simulink model "hw3_model"  (R2024b)
settings: Solver=ode4  StartTime=0.0  StopTime=120.0  FixedStep=0.05  RelTol=1e-3
undefined symbols (not defined in the file): k, L, v, waypoints
settings Model: Creator=Atakan  LastModifiedBy=Atakan

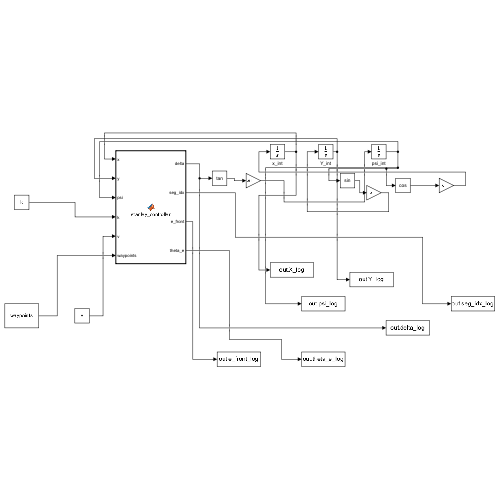
[thumbnail: Simulink's stored preview of the top-level diagram]
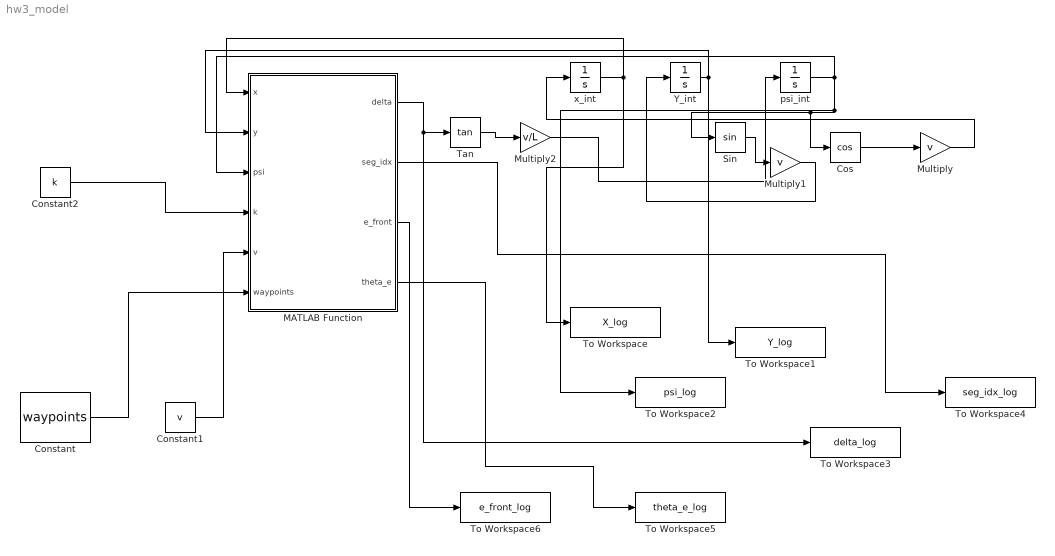
== system hw3_model ==
  Constant : Constant  Value=waypoints
  Constant1 : Constant  Value=v
  Constant2 : Constant  Value=k
  Cos : Trigonometry  Operator=cos
  MATLAB Function : MATLAB Function  TreatAsAtomicUnit=on  SystemSampleTime=0.05
  Multiply : Gain  Gain=v
  Multiply1 : Gain  Gain=v
  Multiply2 : Gain  Gain=v/L
  Sin : Trigonometry
  Tan : Trigonometry  Operator=tan
  To Workspace : ToWorkspace  VariableName=X_log  SaveFormat=Timeseries  SampleTime=-1
  To Workspace1 : ToWorkspace  VariableName=Y_log  SaveFormat=Timeseries  SampleTime=-1
  To Workspace2 : ToWorkspace  VariableName=psi_log  SaveFormat=Timeseries  SampleTime=-1
  To Workspace3 : ToWorkspace  VariableName=delta_log  SaveFormat=Timeseries  SampleTime=-1
  To Workspace4 : ToWorkspace  VariableName=seg_idx_log  SaveFormat=Timeseries  SampleTime=-1
  To Workspace5 : ToWorkspace  VariableName=theta_e_log  SaveFormat=Timeseries  SampleTime=-1
  To Workspace6 : ToWorkspace  VariableName=e_front_log  SaveFormat=Timeseries  SampleTime=-1
  Y_int : Integrator
  psi_int : Integrator  InitialCondition=atan2(5,10)
  x_int : Integrator
  wires:
  psi_int/1 -> To Workspace2/1, Sin/1, Cos/1, MATLAB Function/3(psi)
  Cos/1 -> Multiply/1
  Multiply/1 -> x_int/1
  Sin/1 -> Multiply1/1
  Multiply1/1 -> Y_int/1
  MATLAB Function/1(delta) -> To Workspace3/1, Tan/1
  Tan/1 -> Multiply2/1
  Multiply2/1 -> psi_int/1
  MATLAB Function/2(seg_idx) -> To Workspace4/1
  x_int/1 -> To Workspace/1, MATLAB Function/1(x)
  Y_int/1 -> To Workspace1/1, MATLAB Function/2(y)
  Constant/1 -> MATLAB Function/6(waypoints)
  Constant1/1 -> MATLAB Function/5(v)
  Constant2/1 -> MATLAB Function/4(k)
  MATLAB Function/3(e_front) -> To Workspace6/1
  MATLAB Function/4(theta_e) -> To Workspace5/1

== matlab function hw3_model/MATLAB Function ==
  data: x input; delta output; y input; psi input; k input; v input; waypoints input; seg_idx output; e_front output; theta_e output
function [delta, seg_idx, e_front, theta_e] = stanley_controller(x, y, psi, k, v, waypoints)
% Stanley path tracking controller for front axle reference point
%
% Inputs:
%   x, y       : front axle center position [m]
%   psi        : vehicle heading angle [rad]
%   k          : Stanley gain
%   v          : constant longitudinal velocity [m/s]
%   waypoints  : Nx2 waypoint matrix
%
% Outputs:
%   delta      : steering command [rad]
%   seg_idx    : active segment index
%   e_front    : signed front axle cross-track error [m]
%   theta_e    : heading error [rad]

persistent current_segment

if isempty(current_segment)
    current_segment = 1;
end

N = size(waypoints, 1);

% Limit segment index
if current_segment > N - 1
    current_segment = N - 1;
end

pf = [x; y];

% Current segment
p1 = waypoints(current_segment, :)';
p2 = waypoints(current_segment + 1, :)';

seg_vec = p2 - p1;
seg_len = norm(seg_vec);

if seg_len < 1e-9
    delta = 0;
    seg_idx = current_segment;
    e_front = 0;
    theta_e = 0;
    return;
end

t_hat = seg_vec / seg_len;

% Projection parameter on current segment
rel_vec = pf - p1;
s = dot(rel_vec, t_hat);
progress = s / seg_len;

% Distance to next waypoint
dist_to_next = norm(pf - p2);

% More conservative segment switching
switch_distance = 1.5;

if (progress >= 1.0 || dist_to_next < switch_distance) && current_segment < N - 1
    current_segment = current_segment + 1;

    % Recompute segment after switching
    p1 = waypoints(current_segment, :)';
    p2 = waypoints(current_segment + 1, :)';

    seg_vec = p2 - p1;
    seg_len = norm(seg_vec);
    t_hat = seg_vec / seg_len;

    rel_vec = pf - p1;
    s = dot(rel_vec, t_hat);
end

% Clamp projection onto segment for error calculation
s_clamped = min(max(s, 0), seg_len);
p_proj = p1 + s_clamped * t_hat;

% Path heading
path_yaw = atan2(t_hat(2), t_hat(1));

% Heading error
theta_e = wrapToPiLocal(path_yaw - psi);

% Unit normal vector to the left of path direction
n_hat = [-t_hat(2); t_hat(1)];

% Signed cross-track error
% IMPORTANT:
% Error is defined from vehicle front axle point to projected path point.
% This sign convention makes positive delta steer toward the path.
e_front = dot((p_proj - pf), n_hat);

% Stanley control law
delta_unsat = theta_e + atan2(k * e_front, max(v, 0.1));

% Steering saturation
delta_max = 0.5236;

if delta_unsat > delta_max
    delta = delta_max;
elseif delta_unsat < -delta_max
    delta = -delta_max;
else
    delta = delta_unsat;
end

seg_idx = current_segment;

end


function angle = wrapToPiLocal(angle)

while angle > pi
    angle = angle - 2*pi;
end

while angle < -pi
    angle = angle + 2*pi;
end

end
